simulink model "OffRoadMultibodyStage1_TireDamping_Cz20_20261101"  (R2026a)
settings: Solver=ode15s  StopTime=100  RelTol=2e-3  EnableMultiTasking=on
values from neighbouring files (symbols this model uses):
  goalX = goalPoseWorkflow(1)    [buildCustomPhysicalScenarioModel.m]    (also in correctCustomObstacle3Spawn.m; createScenarioIntegrationTestModel.m = goalPose(1); planAroundConfiguredObstacle.m = originalPath(end,1); restoreRoughTerrainWorkspace.m = goalXY(1))
  goalY = goalPoseWorkflow(2)    [buildCustomPhysicalScenarioModel.m]    (also in correctCustomObstacle3Spawn.m; createScenarioIntegrationTestModel.m = goalPose(2); planAroundConfiguredObstacle.m = originalPath(end,2); restoreRoughTerrainWorkspace.m = goalXY(2))
  obstacle3X = obs(3).centerXY(1)    [buildCustomPhysicalScenarioModel.m]    (also in correctCustomObstacle3Spawn.m = o3.centerXY(1); createScenarioIntegrationTestModel.m = obstacleXs(3); restoreRoughTerrainWorkspace.m = obstacleXs(3); runCustomObstacle5DelayedAblation32s.m = double(obs(3).centerXY(1)))
  obstacle3Y = obs(3).centerXY(2)    [buildCustomPhysicalScenarioModel.m]    (also in correctCustomObstacle3Spawn.m = o3.centerXY(2); createScenarioIntegrationTestModel.m = obstacleYs(3); restoreRoughTerrainWorkspace.m = obstacleYs(3); runCustomObstacle5DelayedAblation32s.m = double(obs(3).centerXY(2)))
  obstacleSpawnTime = [obstacleSpawnTime nan(1,4)]    [buildCustomPhysicalScenarioModel.m]    (also in correctCustomObstacle3Spawn.m = [[obs.spawnTime] nan(1,4)]; createScenarioIntegrationTestModel.m = [obs.spawnTime]; restoreRoughTerrainWorkspace.m = [obs.spawnTime]; runCustomObstacle5DelayedAblation32s.m = [[obs.spawnTime] nan(1,4)])
  obstacleXs = [obstacleXs nan(1,4)]    [buildCustomPhysicalScenarioModel.m]    (also in correctCustomObstacle3Spawn.m = [allCenters(:,1).' nan(1,4)]; createScenarioIntegrationTestModel.m = allCenters(:,1).'; onlineReplanFromPose.m = obstacleXs(valid); onlineReplanFromPoseGeometryAware.m = obstacleXs(valid))
  obstacleYs = [obstacleYs nan(1,4)]    [buildCustomPhysicalScenarioModel.m]    (also in correctCustomObstacle3Spawn.m = [allCenters(:,2).' nan(1,4)]; createScenarioIntegrationTestModel.m = allCenters(:,2).'; onlineReplanFromPose.m = obstacleYs(valid); onlineReplanFromPoseGeometryAware.m = obstacleYs(valid))
  originalPathPadded = [ ... (first row only)    [planAroundConfiguredObstacle.m]
  s = blockNames{k}    [inspectPhysicalScenarioModel.m]    (also in inspectSteeringControllerAndTransferFcn.m = strtrim(s); inspectSteeringJointSignalPath.m = valueToText(v); runCustomSolverProfiler40s.m = profileResult.summary)
  X = X(:)'    [launchElevationTerrainRoverViewer.m]    (also in launchElevationTerrainRoverViewerMultiDynamic.m; launchRoughTerrainScenarioEditor.m = double(evalin('base', 'X')); previewGeometryAwareObstaclePlanner.m = evalin('base','X'))
  Y = Y(:)    [launchElevationTerrainRoverViewer.m]    (also in launchElevationTerrainRoverViewerMultiDynamic.m; launchRoughTerrainScenarioEditor.m = double(evalin('base', 'Y')); previewGeometryAwareObstaclePlanner.m = evalin('base','Y'))
  Z = double(Z_multibody)    [inspectFailureLocation.m]    (also in launchElevationTerrainRoverViewer.m = ZGridSurface.'; launchElevationTerrainRoverViewerMultiDynamic.m = ZGridSurface.'; previewGeometryAwareObstaclePlanner.m = evalin('base','Z'))
libraries: nesl_utility x71, sm_lib x45, slpidlib x1
(part 2 of 2)

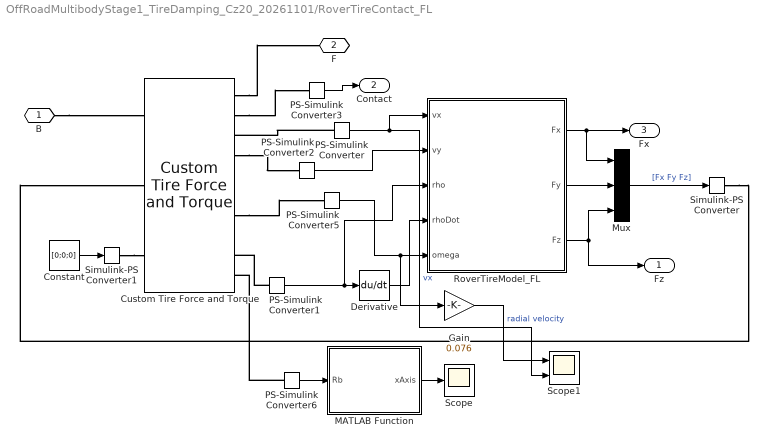
== system OffRoadMultibodyStage1_TireDamping_Cz20_20261101/RoverTireContact_FL ==
  Constant : Constant  Value=[0;0;0]
  Custom Tire Force and Torque : sm_lib/Forces and Torques/Custom Tire Force and Torque  TireRadius=0.076  TireRadiusUnits=m  ContactFrameMethod=WeightedPenetration  SenseContactSignal=on  SenseRelativeLongitudinalVelocity=on  SenseRelativeLateralVelocity=on  SenseYawVelocity=on  SenseCamberAngle=on  SenseCamberVelocity=off  SenseSpinVelocity=on  SenseLoadedRadius=on  SenseRadialDeflection=on  SenseContactBaseRotation=on  SenseContactBaseTranslation=off  SenseContactFollowerRotation=off  SenseContactFollowerTranslation=off
  Derivative : Derivative
  Gain : Gain  Gain=0.076
  MATLAB Function : MATLAB Function  TreatAsAtomicUnit=on
  Mux : Mux  Inputs=3
  PS-Simulink Converter{,1..3,5..6} (6 alike) : nesl_utility/PS-Simulink Converter  PhysicalDomain=network_engine_domain  SubClassName=ps_output  LeftPortType=input  RightPortType=output  PseudoPeriodic=off  Frequencies=[]  VectorFormat=inherit  Unit=inherit  AffineConversion=off
  RoverTireModel_FL : MATLAB Function  TreatAsAtomicUnit=on
  Scope : Scope
      settings: ActiveDisplayYMinimum=-1.8113947831024173  ActiveDisplayYMaximum=2.4644433063735272  DataLoggingVariableName=ScopeData6
  Scope1 : Scope  NumInputPorts=2
      settings: ActiveDisplayYMinimum=-19.842312523626063  ActiveDisplayYMaximum=2.2047013915140066  DataLoggingVariableName=ScopeData16
  Simulink-PS Converter : nesl_utility/Simulink-PS Converter  PhysicalDomain=network_engine_domain  SubClassName=ps_input  LeftPortType=input  RightPortType=output  PseudoPeriodic=off  Frequencies=[]  NoiseDistribution=none  NoiseParameters=[]  Unit=N  AffineConversion=off  FilteringAndDerivatives=provide  SimscapeFilterOrder=1  InputFilterTimeConstant=0.001  UdotUserProvided=0
  Simulink-PS Converter1 : nesl_utility/Simulink-PS Converter  PhysicalDomain=network_engine_domain  SubClassName=ps_input  LeftPortType=input  RightPortType=output  PseudoPeriodic=off  Frequencies=[]  NoiseDistribution=none  NoiseParameters=[]  Unit=N*m  AffineConversion=off  FilteringAndDerivatives=provide  SimscapeFilterOrder=1  InputFilterTimeConstant=0.001  UdotUserProvided=0
  B : PMIOPort  Side=Left
  F : PMIOPort  Port=2  Side=Right
  Fz : Outport
  Contact : Outport  Port=2
  Fx : Outport  Port=3
  wires:
  PS-Simulink Converter2/1 -> RoverTireModel_FL/2(vy)
  RoverTireModel_FL/2(Fy) -> Mux/2
  PS-Simulink Converter1/1 -> RoverTireModel_FL/3(rho), Derivative/1
  Constant/1 -> Simulink-PS Converter1/1
  Mux/1 -> Simulink-PS Converter/1  "[Fx Fy Fz]"
  PS-Simulink Converter/1 -> Scope1/2, RoverTireModel_FL/1(vx)  "vx"
  RoverTireModel_FL/1(Fx) -> Fx/1, Mux/1
  RoverTireModel_FL/3(Fz) -> Fz/1, Mux/3
  PS-Simulink Converter3/1 -> Contact/1
  Derivative/1 -> RoverTireModel_FL/4(rhoDot)
  PS-Simulink Converter5/1 -> Gain/1, RoverTireModel_FL/5(omega)
  PS-Simulink Converter6/1 -> MATLAB Function/1(Rb)
  MATLAB Function/1(xAxis) -> Scope/1
  Gain/1 -> Scope1/1  "radial velocity"
  connections:
  PS-Simulink Converter1/LConn1 -- Custom Tire Force and Torque/RConn9
  Custom Tire Force and Torque/RConn4 -- PS-Simulink Converter2/LConn1
  PS-Simulink Converter/LConn1 -- Custom Tire Force and Torque/RConn3
  Simulink-PS Converter1/RConn1 -- Custom Tire Force and Torque/LConn3
  Simulink-PS Converter/RConn1 -- Custom Tire Force and Torque/LConn2
  Custom Tire Force and Torque/RConn1 -- F/RConn1
  B/RConn1 -- Custom Tire Force and Torque/LConn1
  Custom Tire Force and Torque/RConn2 -- PS-Simulink Converter3/LConn1
  Custom Tire Force and Torque/RConn7 -- PS-Simulink Converter5/LConn1
  PS-Simulink Converter6/LConn1 -- Custom Tire Force and Torque/RConn10

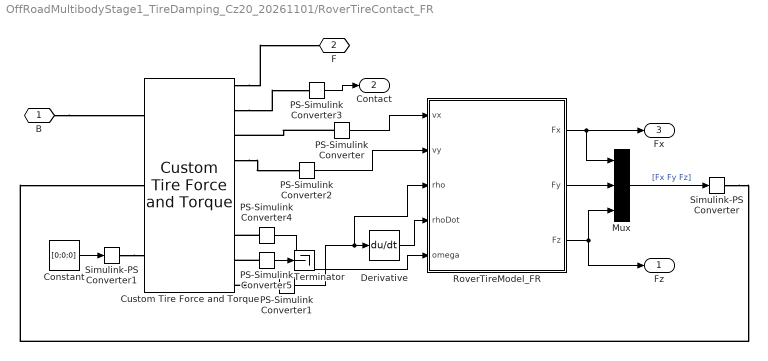
== system OffRoadMultibodyStage1_TireDamping_Cz20_20261101/RoverTireContact_FR ==
  Constant : Constant  Value=[0;0;0]
  Custom Tire Force and Torque : sm_lib/Forces and Torques/Custom Tire Force and Torque  TireRadius=0.076  TireRadiusUnits=m  ContactFrameMethod=WeightedPenetration  SenseContactSignal=on  SenseRelativeLongitudinalVelocity=on  SenseRelativeLateralVelocity=on  SenseYawVelocity=on  SenseCamberAngle=on  SenseCamberVelocity=off  SenseSpinVelocity=on  SenseLoadedRadius=on  SenseRadialDeflection=on  SenseContactBaseRotation=off  SenseContactBaseTranslation=off  SenseContactFollowerRotation=off  SenseContactFollowerTranslation=off
  Derivative : Derivative
  Mux : Mux  Inputs=3
  PS-Simulink Converter{,1..5} (6 alike) : nesl_utility/PS-Simulink Converter  PhysicalDomain=network_engine_domain  SubClassName=ps_output  LeftPortType=input  RightPortType=output  PseudoPeriodic=off  Frequencies=[]  VectorFormat=inherit  Unit=inherit  AffineConversion=off
  RoverTireModel_FR : MATLAB Function  TreatAsAtomicUnit=on
  Simulink-PS Converter : nesl_utility/Simulink-PS Converter  PhysicalDomain=network_engine_domain  SubClassName=ps_input  LeftPortType=input  RightPortType=output  PseudoPeriodic=off  Frequencies=[]  NoiseDistribution=none  NoiseParameters=[]  Unit=N  AffineConversion=off  FilteringAndDerivatives=provide  SimscapeFilterOrder=1  InputFilterTimeConstant=0.001  UdotUserProvided=0
  Simulink-PS Converter1 : nesl_utility/Simulink-PS Converter  PhysicalDomain=network_engine_domain  SubClassName=ps_input  LeftPortType=input  RightPortType=output  PseudoPeriodic=off  Frequencies=[]  NoiseDistribution=none  NoiseParameters=[]  Unit=N*m  AffineConversion=off  FilteringAndDerivatives=provide  SimscapeFilterOrder=1  InputFilterTimeConstant=0.001  UdotUserProvided=0
  Terminator : Terminator
  B : PMIOPort  Side=Left
  F : PMIOPort  Port=2  Side=Right
  Fz : Outport
  Contact : Outport  Port=2
  Fx : Outport  Port=3
  wires:
  PS-Simulink Converter2/1 -> RoverTireModel_FR/2(vy)
  RoverTireModel_FR/2(Fy) -> Mux/2
  PS-Simulink Converter1/1 -> RoverTireModel_FR/3(rho), Derivative/1
  Constant/1 -> Simulink-PS Converter1/1
  Mux/1 -> Simulink-PS Converter/1  "[Fx Fy Fz]"
  PS-Simulink Converter/1 -> RoverTireModel_FR/1(vx)
  RoverTireModel_FR/1(Fx) -> Fx/1, Mux/1
  RoverTireModel_FR/3(Fz) -> Fz/1, Mux/3
  PS-Simulink Converter3/1 -> Contact/1
  Derivative/1 -> RoverTireModel_FR/4(rhoDot)
  PS-Simulink Converter4/1 -> RoverTireModel_FR/5(omega)
  PS-Simulink Converter5/1 -> Terminator/1
  connections:
  PS-Simulink Converter1/LConn1 -- Custom Tire Force and Torque/RConn9
  Custom Tire Force and Torque/RConn4 -- PS-Simulink Converter2/LConn1
  PS-Simulink Converter/LConn1 -- Custom Tire Force and Torque/RConn3
  Simulink-PS Converter1/RConn1 -- Custom Tire Force and Torque/LConn3
  Simulink-PS Converter/RConn1 -- Custom Tire Force and Torque/LConn2
  Custom Tire Force and Torque/RConn1 -- F/RConn1
  B/RConn1 -- Custom Tire Force and Torque/LConn1
  Custom Tire Force and Torque/RConn2 -- PS-Simulink Converter3/LConn1
  PS-Simulink Converter5/LConn1 -- Custom Tire Force and Torque/RConn8
  PS-Simulink Converter4/LConn1 -- Custom Tire Force and Torque/RConn7

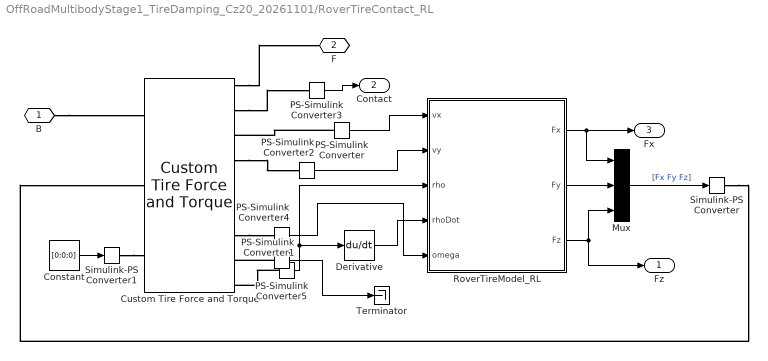
== system OffRoadMultibodyStage1_TireDamping_Cz20_20261101/RoverTireContact_RL ==
  Constant : Constant  Value=[0;0;0]
  Custom Tire Force and Torque : sm_lib/Forces and Torques/Custom Tire Force and Torque  TireRadius=0.076  TireRadiusUnits=m  ContactFrameMethod=WeightedPenetration  SenseContactSignal=on  SenseRelativeLongitudinalVelocity=on  SenseRelativeLateralVelocity=on  SenseYawVelocity=on  SenseCamberAngle=on  SenseCamberVelocity=off  SenseSpinVelocity=on  SenseLoadedRadius=on  SenseRadialDeflection=on  SenseContactBaseRotation=off  SenseContactBaseTranslation=off  SenseContactFollowerRotation=off  SenseContactFollowerTranslation=off
  Derivative : Derivative
  Mux : Mux  Inputs=3
  PS-Simulink Converter{,1..5} (6 alike) : nesl_utility/PS-Simulink Converter  PhysicalDomain=network_engine_domain  SubClassName=ps_output  LeftPortType=input  RightPortType=output  PseudoPeriodic=off  Frequencies=[]  VectorFormat=inherit  Unit=inherit  AffineConversion=off
  RoverTireModel_RL : MATLAB Function  TreatAsAtomicUnit=on
  Simulink-PS Converter : nesl_utility/Simulink-PS Converter  PhysicalDomain=network_engine_domain  SubClassName=ps_input  LeftPortType=input  RightPortType=output  PseudoPeriodic=off  Frequencies=[]  NoiseDistribution=none  NoiseParameters=[]  Unit=N  AffineConversion=off  FilteringAndDerivatives=provide  SimscapeFilterOrder=1  InputFilterTimeConstant=0.001  UdotUserProvided=0
  Simulink-PS Converter1 : nesl_utility/Simulink-PS Converter  PhysicalDomain=network_engine_domain  SubClassName=ps_input  LeftPortType=input  RightPortType=output  PseudoPeriodic=off  Frequencies=[]  NoiseDistribution=none  NoiseParameters=[]  Unit=N*m  AffineConversion=off  FilteringAndDerivatives=provide  SimscapeFilterOrder=1  InputFilterTimeConstant=0.001  UdotUserProvided=0
  Terminator : Terminator
  B : PMIOPort  Side=Left
  F : PMIOPort  Port=2  Side=Right
  Fz : Outport
  Contact : Outport  Port=2
  Fx : Outport  Port=3
  wires:
  PS-Simulink Converter2/1 -> RoverTireModel_RL/2(vy)
  RoverTireModel_RL/2(Fy) -> Mux/2
  PS-Simulink Converter1/1 -> Derivative/1, RoverTireModel_RL/3(rho)
  Constant/1 -> Simulink-PS Converter1/1
  Mux/1 -> Simulink-PS Converter/1  "[Fx Fy Fz]"
  PS-Simulink Converter/1 -> RoverTireModel_RL/1(vx)
  RoverTireModel_RL/1(Fx) -> Fx/1, Mux/1
  RoverTireModel_RL/3(Fz) -> Fz/1, Mux/3
  PS-Simulink Converter3/1 -> Contact/1
  Derivative/1 -> RoverTireModel_RL/4(rhoDot)
  PS-Simulink Converter4/1 -> RoverTireModel_RL/5(omega)
  PS-Simulink Converter5/1 -> Terminator/1
  connections:
  PS-Simulink Converter1/LConn1 -- Custom Tire Force and Torque/RConn9
  Custom Tire Force and Torque/RConn4 -- PS-Simulink Converter2/LConn1
  PS-Simulink Converter/LConn1 -- Custom Tire Force and Torque/RConn3
  Simulink-PS Converter1/RConn1 -- Custom Tire Force and Torque/LConn3
  Simulink-PS Converter/RConn1 -- Custom Tire Force and Torque/LConn2
  Custom Tire Force and Torque/RConn1 -- F/RConn1
  B/RConn1 -- Custom Tire Force and Torque/LConn1
  Custom Tire Force and Torque/RConn2 -- PS-Simulink Converter3/LConn1
  Custom Tire Force and Torque/RConn7 -- PS-Simulink Converter4/LConn1
  PS-Simulink Converter5/LConn1 -- Custom Tire Force and Torque/RConn8

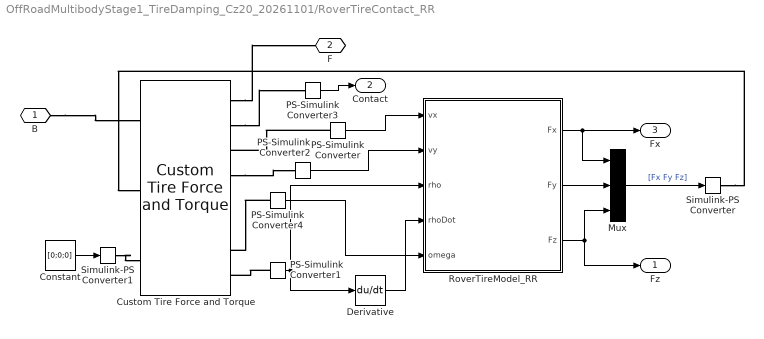
== system OffRoadMultibodyStage1_TireDamping_Cz20_20261101/RoverTireContact_RR ==
  Constant : Constant  Value=[0;0;0]
  Custom Tire Force and Torque : sm_lib/Forces and Torques/Custom Tire Force and Torque  TireRadius=0.076  TireRadiusUnits=m  ContactFrameMethod=WeightedPenetration  SenseContactSignal=on  SenseRelativeLongitudinalVelocity=on  SenseRelativeLateralVelocity=on  SenseYawVelocity=on  SenseCamberAngle=on  SenseCamberVelocity=off  SenseSpinVelocity=on  SenseLoadedRadius=off  SenseRadialDeflection=on  SenseContactBaseRotation=off  SenseContactBaseTranslation=off  SenseContactFollowerRotation=off  SenseContactFollowerTranslation=off
  Derivative : Derivative
  Mux : Mux  Inputs=3
  PS-Simulink Converter{,1..4} (5 alike) : nesl_utility/PS-Simulink Converter  PhysicalDomain=network_engine_domain  SubClassName=ps_output  LeftPortType=input  RightPortType=output  PseudoPeriodic=off  Frequencies=[]  VectorFormat=inherit  Unit=inherit  AffineConversion=off
  RoverTireModel_RR : MATLAB Function  TreatAsAtomicUnit=on
  Simulink-PS Converter : nesl_utility/Simulink-PS Converter  PhysicalDomain=network_engine_domain  SubClassName=ps_input  LeftPortType=input  RightPortType=output  PseudoPeriodic=off  Frequencies=[]  NoiseDistribution=none  NoiseParameters=[]  Unit=N  AffineConversion=off  FilteringAndDerivatives=provide  SimscapeFilterOrder=1  InputFilterTimeConstant=0.001  UdotUserProvided=0
  Simulink-PS Converter1 : nesl_utility/Simulink-PS Converter  PhysicalDomain=network_engine_domain  SubClassName=ps_input  LeftPortType=input  RightPortType=output  PseudoPeriodic=off  Frequencies=[]  NoiseDistribution=none  NoiseParameters=[]  Unit=N*m  AffineConversion=off  FilteringAndDerivatives=provide  SimscapeFilterOrder=1  InputFilterTimeConstant=0.001  UdotUserProvided=0
  B : PMIOPort  Side=Left
  F : PMIOPort  Port=2  Side=Right
  Fz : Outport
  Contact : Outport  Port=2
  Fx : Outport  Port=3
  wires:
  PS-Simulink Converter2/1 -> RoverTireModel_RR/2(vy)
  RoverTireModel_RR/2(Fy) -> Mux/2
  PS-Simulink Converter1/1 -> RoverTireModel_RR/3(rho), Derivative/1
  Constant/1 -> Simulink-PS Converter1/1
  Mux/1 -> Simulink-PS Converter/1  "[Fx Fy Fz]"
  PS-Simulink Converter/1 -> RoverTireModel_RR/1(vx)
  RoverTireModel_RR/1(Fx) -> Mux/1, Fx/1
  RoverTireModel_RR/3(Fz) -> Fz/1, Mux/3
  PS-Simulink Converter3/1 -> Contact/1
  Derivative/1 -> RoverTireModel_RR/4(rhoDot)
  PS-Simulink Converter4/1 -> RoverTireModel_RR/5(omega)
  connections:
  PS-Simulink Converter1/LConn1 -- Custom Tire Force and Torque/RConn8
  Custom Tire Force and Torque/RConn4 -- PS-Simulink Converter2/LConn1
  PS-Simulink Converter/LConn1 -- Custom Tire Force and Torque/RConn3
  Simulink-PS Converter1/RConn1 -- Custom Tire Force and Torque/LConn3
  Simulink-PS Converter/RConn1 -- Custom Tire Force and Torque/LConn2
  Custom Tire Force and Torque/RConn1 -- F/RConn1
  B/RConn1 -- Custom Tire Force and Torque/LConn1
  Custom Tire Force and Torque/RConn2 -- PS-Simulink Converter3/LConn1
  PS-Simulink Converter4/LConn1 -- Custom Tire Force and Torque/RConn7

== matlab function OffRoadMultibodyStage1_TireDamping_Cz20_20261101/LongitudinalVelocity ==
  data: vx input; vLong output; vy input; q0 input; q1 input; q2 input; q3 input
function vLong = LongitudinalVelocity(vx, vy, q0, q1, q2, q3)
%#codegen

% Rover yaw from scalar-first quaternion [q0 q1 q2 q3]
yaw = atan2( ...
    2*(q0*q3 + q1*q2), ...
    1 - 2*(q2*q2 + q3*q3));

% World-frame velocity projected onto the rover's forward axis
vLong = vx*cos(yaw) + vy*sin(yaw);

end

== matlab function OffRoadMultibodyStage1_TireDamping_Cz20_20261101/ObstacleSensorLogic ==
  settings: updateMethod=DISCRETE  sampleTime=0.02
  data: x input; detected output; newDetection output; y input; q0 input; q1 input; q2 input; q3 input; environmentXs input; environmentYs input; detectedX output; detectedY output
function [detected, newDetection, detectedX, detectedY] = ...
    fcn(x, y, q0, q1, q2, q3, environmentXs, environmentYs)

persistent seenObstacle anyDetected

if isempty(anyDetected)
    seenObstacle = false(1, numel(environmentXs));
    anyDetected = false;
end

% Virtual forward sensor
sensorRange = 18.0;
halfFOV = pi;  % 45 degrees on either side

% Default: no new obstacle detected in this sample
newDetection = 0;
detectedX = 0;
detectedY = 0;

% Rover yaw from quaternion
yaw = atan2(2*(q0*q3 + q1*q2), ...
            1 - 2*(q2*q2 + q3*q3));

bestIndex = 0;
bestRange = inf;

% Find the nearest previously unseen obstacle in view
for k = 1:numel(environmentXs)

    if seenObstacle(k)
        continue;
    end

    dx = environmentXs(k) - x;
    dy = environmentYs(k) - y;

    range = hypot(dx, dy);
    bearing = atan2(dy, dx) - yaw;
    bearing = atan2(sin(bearing), cos(bearing));

    if range <= sensorRange && ...
            abs(bearing) <= halfFOV && range < bestRange
        bestIndex = k;
        bestRange = range;
    end
end

% Emit a pulse for each newly detected obstacle
if bestIndex > 0
    seenObstacle(bestIndex) = true;
    anyDetected = true;

    newDetection = 1;
    detectedX = environmentXs(bestIndex);
    detectedY = environmentYs(bestIndex);
end

% Keep the route switch on the replacement route after first detection
detected = double(anyDetected);

end

== matlab function OffRoadMultibodyStage1_TireDamping_Cz20_20261101/OnlineReplanManager ==
  settings: updateMethod=DISCRETE  sampleTime=0.02
  data: x input; route output; y input; newDetection input; goalX input; goalY input; detectedX input; detectedY input; routeReady output; replanEvent output; replanStartX output; replanStartY output
function [route, routeReady, replanEvent, replanStartX, replanStartY] = ...
    fcn(x, y, newDetection, goalX, goalY, detectedX, detectedY)
coder.extrinsic('onlineReplanFromPoseGeometryAware');
persistent routeStored routeReadyState
persistent knownXs knownYs knownCount waitCount pending
persistent startXStored startYStored
maxWaypoints = 100;
maxObstacles = 10;
settleSteps = 10; % 0.2 s at 0.02 s sample time
if isempty(routeReadyState)
    routeStored = zeros(maxWaypoints,2);
    routeReadyState = false;
    knownXs = nan(1,maxObstacles);
    knownYs = nan(1,maxObstacles);
    knownCount = 0; waitCount = 0; pending = false;
    startXStored = 0; startYStored = 0;
end
replanEvent = 0;
if newDetection >= 0.5
    duplicate = false;
    for k = 1:knownCount
        if hypot(knownXs(k)-detectedX, knownYs(k)-detectedY) < 0.25
            duplicate = true; break;
        end
    end
    if ~duplicate && knownCount < maxObstacles
        knownCount = knownCount + 1;
        knownXs(knownCount) = detectedX; knownYs(knownCount) = detectedY;
        pending = true;
    end
    waitCount = 0;
elseif pending
    waitCount = waitCount + 1;
end
if pending && waitCount >= settleSteps
    candidateRoute = zeros(maxWaypoints,2);
    candidateRoute = onlineReplanFromPoseGeometryAware( ...
        [x y], [goalX goalY], knownXs(1:knownCount), ...
        knownYs(1:knownCount), 3.5, maxWaypoints);
    routeStored = candidateRoute;
    startXStored = routeStored(1,1); startYStored = routeStored(1,2);
    routeReadyState = true; pending = false; waitCount = 0;
    replanEvent = 1;
end
route = routeStored; routeReady = double(routeReadyState);
replanStartX = startXStored; replanStartY = startYStored;
end

== matlab function OffRoadMultibodyStage1_TireDamping_Cz20_20261101/DynamicObstacleEnvironment ==
  data: t input; environmentXs output; knownXs input; knownYs input; obstacle3X input; obstacle3Y input; spawnTime input; environmentYs output
function [environmentXs, environmentYs] = ...
    fcn(t, knownXs, knownYs, obstacle3X, obstacle3Y, spawnTime)
% Fixed capacity: up to 10 scenario obstacles.
% NaN spawnTime means static from t=0; finite spawnTime activates by time t.
maxScenarioObstacles = 10;
environmentXs = nan(1,maxScenarioObstacles);
environmentYs = nan(1,maxScenarioObstacles);
for k = 1:maxScenarioObstacles
    if numel(knownXs) >= k && numel(knownYs) >= k && numel(spawnTime) >= k
        tk = spawnTime(k);
        if isnan(tk) || t >= tk
            environmentXs(k) = knownXs(k);
            environmentYs(k) = knownYs(k);
        end
    end
end
end

== matlab function OffRoadMultibodyStage1_TireDamping_Cz20_20261101/RoverTireContact_FR/RoverTireModel_FR ==
  data: vx input; Fx output; vy input; rho input; rhoDot input; Fy output; Fz output; omega input
function [Fx,Fy,Fz] = RoverTireModel_FR(vx,vy,rho,rhoDot,omega)

kz = 5000;
cz = 20;
mu = 0.7;

R  = 0.076;
Cx = 300;

Fz = max(0, kz*rho + cz*rhoDot);

vSlip = R*omega - vx;
Fx = Cx*vSlip;
Fy = -1500*vy;

Fx = max(-mu*Fz, min(mu*Fz, Fx));
Fy = max(-mu*Fz, min(mu*Fz, Fy));

end

== matlab function OffRoadMultibodyStage1_TireDamping_Cz20_20261101/RoverTireContact_FL/RoverTireModel_FL ==
  data: vx input; Fx output; vy input; rho input; rhoDot input; omega input; Fy output; Fz output
function [Fx,Fy,Fz] = RoverTireModel_FL(vx,vy,rho,rhoDot,omega)

kz = 5000;
cz = 20;
mu = 0.7;

R  = 0.076;   % Wheel radius (m)
Cx = 300;     % Initial longitudinal slip coefficient

Fz = max(0, kz*rho + cz*rhoDot);

% Longitudinal slip velocity due to wheel rotation
vSlip = R*omega - vx;

% Traction force generated by wheel slip
Fx = Cx*vSlip;

% Retain the simplified lateral resistance
Fy = -1500*vy;

% Limit tangential forces by available friction
Fx = max(-mu*Fz, min(mu*Fz, Fx));
Fy = max(-mu*Fz, min(mu*Fz, Fy));

end

== matlab function OffRoadMultibodyStage1_TireDamping_Cz20_20261101/RoverTireContact_RL/RoverTireModel_RL ==
  data: vx input; Fx output; vy input; rho input; Fy output; Fz output; rhoDot input; omega input
function [Fx,Fy,Fz] = RoverTireModel_RL(vx,vy,rho,rhoDot,omega)

kz = 5000;
cz = 0;
mu = 0.7;

R  = 0.076;
Cx = 300;

Fz = max(0, kz*rho + cz*rhoDot);

vSlip = R*omega - vx;
Fx = Cx*vSlip;
Fy = -1500*vy;

Fx = max(-mu*Fz, min(mu*Fz, Fx));
Fy = max(-mu*Fz, min(mu*Fz, Fy));

end

== matlab function OffRoadMultibodyStage1_TireDamping_Cz20_20261101/RoverTireContact_RR/RoverTireModel_RR ==
  data: vx input; Fx output; vy input; rho input; Fy output; Fz output; rhoDot input; omega input
function [Fx,Fy,Fz] = RoverTireModel_RR(vx,vy,rho,rhoDot,omega)

kz = 5000;
cz = 0;
mu = 0.7;

R  = 0.076;
Cx = 300;

Fz = max(0, kz*rho + cz*rhoDot);


vSlip = R*omega - vx;
Fx = Cx*vSlip;
Fy = -1500*vy;

Fx = max(-mu*Fz, min(mu*Fz, Fx));
Fy = max(-mu*Fz, min(mu*Fz, Fy));

end

== matlab function OffRoadMultibodyStage1_TireDamping_Cz20_20261101/RoverTireContact_FL/MATLAB Function ==
  data: Rb input; xAxis output
function xAxis = contactXAxisWorld(Rb)

xAxis = Rb(:,1);

end

== matlab function OffRoadMultibodyStage1_TireDamping_Cz20_20261101/AckermannSteering ==
  data: delta input; deltaFL output; deltaFR output
function [deltaFL, deltaFR] = AckermannSteering(delta)

L = 1.115;  % Wheelbase (m)
T = 0.920;  % Front track width (m)

tanDelta = tan(delta);

deltaFL = atan(tanDelta / ...
    (1 - (T/(2*L))*tanDelta));

deltaFR = atan(tanDelta / ...
    (1 + (T/(2*L))*tanDelta));

end

== matlab function OffRoadMultibodyStage1_TireDamping_Cz20_20261101/PurePursuitController ==
  data: x input; steerCmd output; y input; q0 input; q1 input; q2 input; q3 input; wp input; speedRef output
function [steerCmd, speedRef] = PurePursuitController( ...
    x, y, q0, q1, q2, q3, wp)
%#codegen

wheelBase = 1.115;    % Wheelbase (m)
lookahead = 1.2;      % Lookahead distance (m)
maxSteer = 0.45;      % Steering limit (rad)

baseSpeed = 1.5;      % Increased straight-line speed (m/s)
minSpeed = 0.6;       % Minimum reference speed during sharp turns

speedRef = baseSpeed;
steerCmd = 0;

n = size(wp,1);
if n < 2
    return;
end

% Quaternion is scalar-first: [q0 q1 q2 q3]
yaw = atan2( ...
    2*(q0*q3 + q1*q2), ...
    1 - 2*(q2*q2 + q3*q3));

% Find the closest projection onto the waypoint polyline.
bestDist2 = inf;
nearestS = 0;
cumulativeS = 0;

for i = 1:n-1
    x1 = wp(i,1);
    y1 = wp(i,2);
    dxSeg = wp(i+1,1) - x1;
    dySeg = wp(i+1,2) - y1;
    segLen2 = dxSeg*dxSeg + dySeg*dySeg;
    segLen = sqrt(segLen2);

    if segLen2 > 1e-12
        t = ((x-x1)*dxSeg + (y-y1)*dySeg)/segLen2;
        t = min(1, max(0, t));

        projX = x1 + t*dxSeg;
        projY = y1 + t*dySeg;

        dist2 = (x-projX)^2 + (y-projY)^2;

        if dist2 < bestDist2
            bestDist2 = dist2;
            nearestS = cumulativeS + t*segLen;
        end
    end

    cumulativeS = cumulativeS + segLen;
end

% Total path length and lookahead target distance.
totalLength = cumulativeS;
targetS = min(nearestS + lookahead, totalLength);

% Interpolate the target point along the polyline.
cumulativeS = 0;
targetX = wp(n,1);
targetY = wp(n,2);

for i = 1:n-1
    x1 = wp(i,1);
    y1 = wp(i,2);
    dxSeg = wp(i+1,1) - x1;
    dySeg = wp(i+1,2) - y1;
    segLen = sqrt(dxSeg*dxSeg + dySeg*dySeg);

    if targetS <= cumulativeS + segLen || i == n-1
        if segLen > 1e-9
            t = (targetS-cumulativeS)/segLen;
            t = min(1, max(0, t));

            targetX = x1 + t*dxSeg;
            targetY = y1 + t*dySeg;
        else
            targetX = wp(i+1,1);
            targetY = wp(i+1,2);
        end
        break;
    end

    cumulativeS = cumulativeS + segLen;
end

% Pure Pursuit steering law.
dxTarget = targetX - x;
dyTarget = targetY - y;
Ld = sqrt(dxTarget*dxTarget + dyTarget*dyTarget);

if Ld > 1e-6
    alpha = atan2(dyTarget, dxTarget) - yaw;
    alpha = atan2(sin(alpha), cos(alpha));

    steerCmd = atan(2*wheelBase*sin(alpha)/Ld);
    steerCmd = min(max(steerCmd, -maxSteer), maxSteer);
end
% Reduce speed as the steering demand increases
steerRatio = min(abs(steerCmd)/maxSteer, 1);

speedRef = baseSpeed ...
    - (baseSpeed - minSpeed)*steerRatio^2;

end

== matlab function OffRoadMultibodyStage1_TireDamping_Cz20_20261101/GoalStopLogic ==
  settings: updateMethod=DISCRETE  sampleTime=0.02
  data: x input; vCmd output; y input; vRef input; goalX input; goalY input

function vCmd = fcn(x, y, vRef, goalX, goalY)

persistent goalReached

if isempty(goalReached)
    goalReached = false;
end

d = hypot(x - goalX, y - goalY);

% Goal approach parameters
stopRadius = 0.15;
crawlRadius = 1.0;
slowdownDistance = 4.0;
minimumScale = 0.60;
terminalScale = 0.06;

% Latch the stopped state at the destination
if d <= stopRadius
    goalReached = true;
end

if goalReached
    vCmd = 0;

else
    if d >= slowdownDistance
        scale = 1.0;

    elseif d >= crawlRadius
        scale = minimumScale + ...
            (1.0 - minimumScale) * ...
            (d - crawlRadius) / ...
            (slowdownDistance - crawlRadius);

    else
        scale = minimumScale * ...
            (d - stopRadius) / ...
            (crawlRadius - stopRadius);

        % Maintain a minimum crawl command
        scale = max(scale, terminalScale);
    end

    vCmd = vRef * scale;
end

end
